simulink model "inverted_spherical_pendulum_lqr"  (R2026b)
settings: Solver=ode45  StopTime=15  MaxStep=0.01  RelTol=1e-09  AbsTol=1e-11
values from neighbouring files (symbols this model uses):
  K = controller.K    [build_simulink_model.m]
  maximum_force = controller.maximum_force    [build_simulink_model.m]
  z0 = reference.states(1,:)'    [build_simulink_model.m]
undefined symbols (not defined in the file or in its folder): g, L, m, M
settings Model: Creator=sahil  LastModifiedBy=sahil

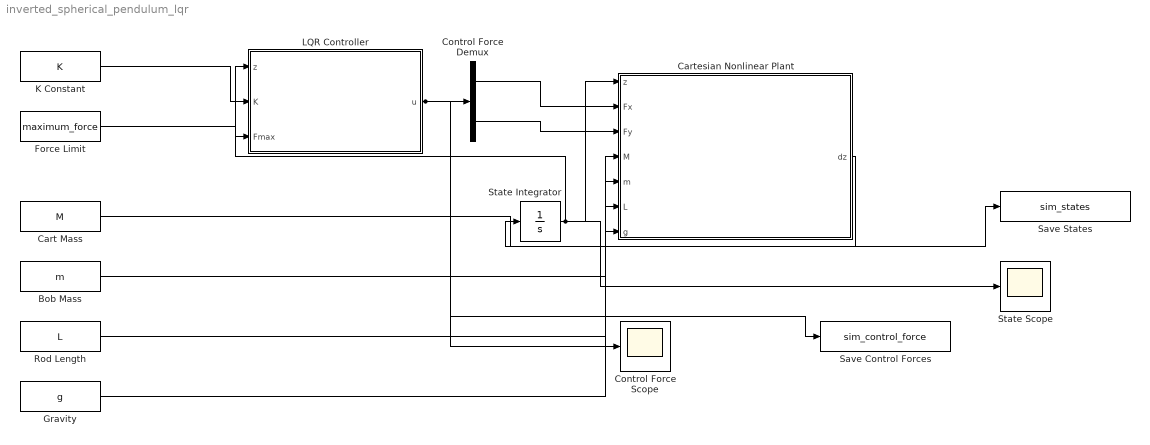
== system inverted_spherical_pendulum_lqr ==
  Bob Mass : Constant  Value=m
  Cart Mass : Constant  Value=M
  Cartesian Nonlinear Plant : MATLAB Function  TreatAsAtomicUnit=on
  Control Force Demux : Demux  Outputs=2
  Control Force Scope : Scope
  Force Limit : Constant  Value=maximum_force
  Gravity : Constant  Value=g
  K Constant : Constant  Value=K
  LQR Controller : MATLAB Function  TreatAsAtomicUnit=on
  Rod Length : Constant  Value=L
  Save Control Forces : ToWorkspace  VariableName=sim_control_force  SaveFormat=Timeseries  SampleTime=-1
  Save States : ToWorkspace  VariableName=sim_states  SaveFormat=Timeseries  SampleTime=-1
  State Integrator : Integrator  InitialCondition=z0
  State Scope : Scope
  wires:
  State Integrator/1 -> LQR Controller/1(z), Cartesian Nonlinear Plant/1(z), Save States/1, State Scope/1
  K Constant/1 -> LQR Controller/2(K)
  Force Limit/1 -> LQR Controller/3(Fmax)
  LQR Controller/1(u) -> Control Force Demux/1, Save Control Forces/1, Control Force Scope/1
  Control Force Demux/1 -> Cartesian Nonlinear Plant/2(Fx)
  Control Force Demux/2 -> Cartesian Nonlinear Plant/3(Fy)
  Cart Mass/1 -> Cartesian Nonlinear Plant/4(M)
  Bob Mass/1 -> Cartesian Nonlinear Plant/5(m)
  Rod Length/1 -> Cartesian Nonlinear Plant/6(L)
  Gravity/1 -> Cartesian Nonlinear Plant/7(g)
  Cartesian Nonlinear Plant/1(dz) -> State Integrator/1

== matlab function inverted_spherical_pendulum_lqr/Cartesian Nonlinear Plant ==
  data: z input; dz output; Fx input; Fy input; M input; m input; L input; g input
function dz = cartesian_plant(z,Fx,Fy,M,m,L,g)
% Nonlinear Cartesian constrained pendulum dynamics

% Generalized coordinates and velocities
x = z(1);
y = z(2);
X = z(3);
Y = z(4);
Z = z(5);

dx = z(6);
dy = z(7);
dX = z(8);
dY = z(9);
dZ = z(10);

% Relative bob position and velocity
r = [X-x; Y-y; Z];
vrel = [dX-dx; dY-dy; dZ];

% Correct 1-by-5 constraint Jacobian
J = [-r(1),-r(2),r(1),r(2),r(3)];

% Generalized mass matrix
D = diag([M,M,m,m,m]);

% Applied generalized forces
Q = [Fx;Fy;0;0;-m*g];

% Acceleration-level rod constraint
constraintAcceleration = -dot(vrel,vrel);

% Lagrange multiplier system
A = [D,-J';J,0];
b = [Q;constraintAcceleration];
solution = A\b;

% Generalized accelerations
qdd = solution(1:5);

% Return ten state derivatives
dz = [dx;dy;dX;dY;dZ;qdd];
end

== matlab function inverted_spherical_pendulum_lqr/LQR Controller ==
  data: z input; u output; K input; Fmax input
function u = lqr_controller(z,K,Fmax)
% Two-axis LQR controller
% Plant state: [x;y;X;Y;Z;dx;dy;dX;dY;dZ]

xi = z(3)-z(1);
eta = z(4)-z(2);
dxi = z(8)-z(6);
deta = z(9)-z(7);

s = [z(1); z(2); xi; eta; ...
     z(6); z(7); dxi; deta];

u = -K*s;

u(1) = min(max(u(1),-Fmax),Fmax);
u(2) = min(max(u(2),-Fmax),Fmax);
end
